simulink model "motion_controller_single"  (R2025a)
settings: configuration reference "AMCBLDC_Configuration" (kept outside this file)
undefined symbols (not defined in the file): AmcbldcInitConf, Ts_Supervision
settings Model: DataDictionary=amcbldc.sldd  Creator=mfussi  LastModifiedBy=mfussi
settings ConfigSetRef: SourceName=AMCBLDC_Configuration

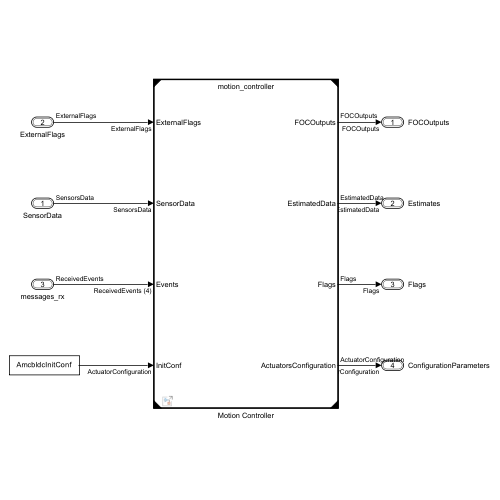
[thumbnail: Simulink's stored preview of the top-level diagram]
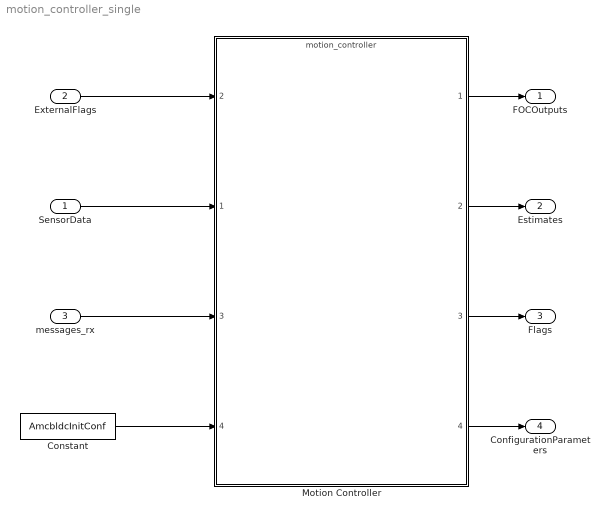
== system motion_controller_single ==
  SensorData : Inport  OutDataTypeStr=Bus: SensorsData  PortDimensions=1  BusOutputAsStruct=on
  ExternalFlags : Inport  Port=2  OutDataTypeStr=Bus: ExternalFlags  BusOutputAsStruct=on
  messages_rx : Inport  Port=3  OutDataTypeStr=Bus: ReceivedEvents  BusOutputAsStruct=on
  Constant : Constant  Value=AmcbldcInitConf  OutDataTypeStr=Bus: ActuatorConfiguration  SampleTime=Ts_Supervision
  Motion Controller : ModelReference  ModelNameDialog=motion_controller.slx  ModelReferenceVersion=5.2
      settings: PortSchema="{\"entries\":[{\"content\":{\"sides\":[{\"content\":{\"connectorIds\":[\"In2\",\"In1\",\"In3\",\"In4\"]},\"type\":\"ConnectorPlacement.EquallySpacedRectSide\",\"uuid\":\"379a1b60-57a2-4ccb-a061-d06c9ad096ee\"},{\"content\":{\"connectorIds\":[\"Out1\",\"Out2\",\"Out3\",\"Out4\"],\"side\":\"RIGHT\"},\"type\":\"ConnectorPlacement.EquallySpacedRectSide\",\"uuid\":\"27b3d028-7796-406c-a973-a0b783b604b2\"},{\"content\":{\"side\":\"TOP\"},\"type\":\"ConnectorPlacement.EquallySpacedRectSide\",\"uuid\":\"38e048f9-e5c6-4a39-8bca-9fbf31731ae5\"}]},\"type\":\"ConnectorPlacement.EquallySpacedConnector\",\"uuid\":\"97b4f620-742c-4215-a432-9dc15dd496c6\"}],\"packageUris\":[\"http://schema.mathworks.com/mf0/Connector/R2020b\"],\"version\":\"1.0\"}"
  FOCOutputs : Outport  OutDataTypeStr=Bus: FOCOutputs  PortDimensions=1  BusOutputAsStruct=on
  Estimates : Outport  Port=2  OutDataTypeStr=Bus: EstimatedData  PortDimensions=1  BusOutputAsStruct=on
  Flags : Outport  Port=3  OutDataTypeStr=Bus: Flags  PortDimensions=1  BusOutputAsStruct=on
  ConfigurationParameters : Outport  Port=4  OutDataTypeStr=Bus: ActuatorConfiguration  PortDimensions=1  BusOutputAsStruct=on
  wires:
  messages_rx/1 -> Motion Controller/3
  Motion Controller/1 -> FOCOutputs/1
  SensorData/1 -> Motion Controller/1
  Motion Controller/4 -> ConfigurationParameters/1
  ExternalFlags/1 -> Motion Controller/2
  Motion Controller/3 -> Flags/1
  Motion Controller/2 -> Estimates/1
  Constant/1 -> Motion Controller/4
